simulink model "AFC_FFNN_trainbfg_15_15_15_15_Nor_July_15"  (R2021a)
settings: Solver=ode15s  StartTime=0.0  StopTime=T  MaxStep=.01  RelTol=1e-3
undefined symbols (not defined in the file): AF_sensor_tol, fault_time, fuel_inj_tol, kappa_tol, MAF_sensor_tol, pump_tol, tau_ww_tol, x_gain, x_offset, y_gain, y_offset
libraries: neural x66
(part 3 of 3)

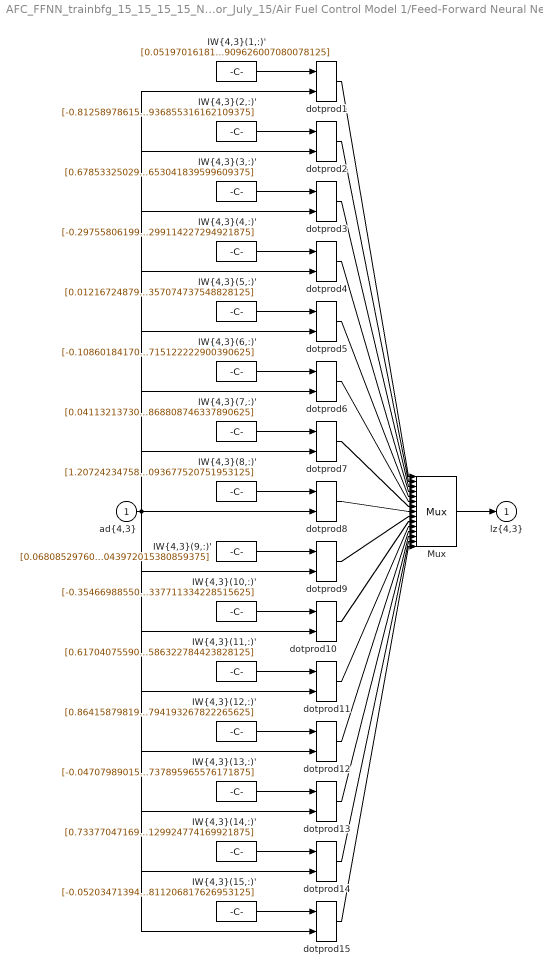
== system AFC_FFNN_trainbfg_15_15_15_15_Nor_July_15/Air Fuel Control Model 1/Feed-Forward Neural Network/Layer 4/LW{4,3} ==
  "ad{4,3}" : Inport  PortDimensions=15
      mask Display: e = 0.06;c1 = [120 230 180]/255;c2 = ([120 230 180]+0)/(256+128);c3 = ([120 230 180]+128)/(256+128);patch([0 1 1 0],[0 0 1 1],c1);patch([0 1 1 1-e 1-e 0+e],[0 0 1 1-e 0+e 0+e],c2);patch([0 0 1 1-e 0+e 0+e],[0 1 1 1-e 1-e 0+e],c3);plot([0 1 1 0 0],[0 0 1 1 0]);
  "IW{4,3}(1,:)'" : Constant  Value=[0.051970161810708959126969830322195775806903839111328125;-0.126328957419962417674241805798374116420745849609375;0.9965377844405078899825412008794955909252166748046875;0.1675357955800376164035014880937524139881134033203125;0.404152985833085953704113535422948189079761505126953125;0.86478973592762808930700657583656720817089080810546875;0.518227264629068873347250701044686138629913330078125;0.2715980210299460129164117461186833679676055908203125;-0.651185893458846809522810872294940054416656494140625;0.319204255476944143143924748073914088308811187744140625;-0.2569115041239822261331937625072896480560302734375;0.057105623983778171226521891412630793638527393341064453125;0.1070777617804902492881780062816687859594821929931640625;-0.82642827178341027316577083183801732957363128662109375;-0.0287179233202064232433059487448190338909626007080078125]
      mask Display: e = 0.06;c1 = [120 150 230]/255;c2 = ([120 150 230]+0)/383;c3 = ([120 150 230]+128)/383;patch([0 1 1 0],[0 0 1 1],c1);patch([0 1 1 1-e 1-e 0+e],[0 0 1 1-e 0+e 0+e],c2);patch([0 0 1 1-e 0+e 0+e],[0 1 1 1-e 1-e 0+e],c3);plot([0 1 1 0 0],[0 0 1 1 0]);disp('weights');
  "IW{4,3}(10,:)'" : Constant  Value=[-0.354669885508523241579581508631235919892787933349609375;-0.77194952346326062286863134431769140064716339111328125;-0.81601175837494732689947340986691415309906005859375;0.379241236877119636261568302870728075504302978515625;-0.3569337623701613892990280874073505401611328125;-0.792692853946006525944767417968250811100006103515625;-0.14953643024327778476845196564681828022003173828125;-0.0850888851491766740053890316630713641643524169921875;-0.9650803191481467369072788642370142042636871337890625;0.405282382043266498072853210032917559146881103515625;0.49853527113881723753507912988425232470035552978515625;0.271502161657881657674806774593889713287353515625;0.3751637008352275426403821256826631724834442138671875;0.8806065157679683341740428659250028431415557861328125;-0.59715081395340219305722939679981209337711334228515625]
      mask Display: e = 0.06;c1 = [120 150 230]/255;c2 = ([120 150 230]+0)/383;c3 = ([120 150 230]+128)/383;patch([0 1 1 0],[0 0 1 1],c1);patch([0 1 1 1-e 1-e 0+e],[0 0 1 1-e 0+e 0+e],c2);patch([0 0 1 1-e 0+e 0+e],[0 1 1 1-e 1-e 0+e],c3);plot([0 1 1 0 0],[0 0 1 1 0]);disp('weights');
  "IW{4,3}(11,:)'" : Constant  Value=[0.617040755904621818217492545954883098602294921875;0.700604235086529580911474113236181437969207763671875;0.511371924663512888997729533002711832523345947265625;0.08963480551315772260068115429021418094635009765625;-0.165964035301581269710169408426736481487751007080078125;0.5031390236482307098953015156439505517482757568359375;0.6633082060229267273854247832787223160266876220703125;-0.709798207981374940089835945400409400463104248046875;0.831096977986841789487471032771281898021697998046875;-0.4122922604000514024136236912454478442668914794921875;-0.0723067339924330365619198346394114196300506591796875;-0.376003397439505893107281053744372911751270294189453125;0.1695995889177781823509150171958026476204395294189453125;0.90183804417739477088389321579597890377044677734375;-1.10240234673867565362570530851371586322784423828125]
      mask Display: e = 0.06;c1 = [120 150 230]/255;c2 = ([120 150 230]+0)/383;c3 = ([120 150 230]+128)/383;patch([0 1 1 0],[0 0 1 1],c1);patch([0 1 1 1-e 1-e 0+e],[0 0 1 1-e 0+e 0+e],c2);patch([0 0 1 1-e 0+e 0+e],[0 1 1 1-e 1-e 0+e],c3);plot([0 1 1 0 0],[0 0 1 1 0]);disp('weights');
  "IW{4,3}(12,:)'" : Constant  Value=[0.86415879819654961568886619716067798435688018798828125;0.1203834479508809618408804453792981803417205810546875;0.133982984467660326544091731193475425243377685546875;-0.0193712548926814331906598454224877059459686279296875;-0.1402303904538838852378290766864665783941745758056640625;1.0897626729878930884609644635929726064205169677734375;0.67839995473971459460926780593581497669219970703125;-0.7508734295524204238603260819218121469020843505859375;0.0334637355957545512552542277262546122074127197265625;0.87659168440380941245138046724605374038219451904296875;-0.980282012415287784534712045569904148578643798828125;0.8080715194356573594092196799465455114841461181640625;-0.76798820148797342088897721623652614653110504150390625;-0.313277713257333612073551876164856366813182830810546875;0.35824559123448074249296269044862128794193267822265625]
      mask Display: e = 0.06;c1 = [120 150 230]/255;c2 = ([120 150 230]+0)/383;c3 = ([120 150 230]+128)/383;patch([0 1 1 0],[0 0 1 1],c1);patch([0 1 1 1-e 1-e 0+e],[0 0 1 1-e 0+e 0+e],c2);patch([0 0 1 1-e 0+e 0+e],[0 1 1 1-e 1-e 0+e],c3);plot([0 1 1 0 0],[0 0 1 1 0]);disp('weights');
  "IW{4,3}(13,:)'" : Constant  Value=[-0.04707989015845824576356193347237422131001949310302734375;-0.74905307149987765402698869365849532186985015869140625;0.5757676864781038350571407136158086359500885009765625;0.71306953158993646724184145568870007991790771484375;-0.5913842257991495099389567258185707032680511474609375;-0.37587419944126232440595458683674223721027374267578125;-0.336733940480412829998613233328796923160552978515625;-0.004068794637174466544138340395875275135040283203125;0.0693886439127837650886476694722659885883331298828125;0.05129647141780004082622923533563152886927127838134765625;-0.0307644877411348029172533102837405749596655368804931640625;-0.334572257247817306247128499308018945157527923583984375;0.2420501582242300664393752640535240061581134796142578125;-0.77793738892486985481156125388224609196186065673828125;1.190993380582610949858235471765510737895965576171875]
      mask Display: e = 0.06;c1 = [120 150 230]/255;c2 = ([120 150 230]+0)/383;c3 = ([120 150 230]+128)/383;patch([0 1 1 0],[0 0 1 1],c1);patch([0 1 1 1-e 1-e 0+e],[0 0 1 1-e 0+e 0+e],c2);patch([0 0 1 1-e 0+e 0+e],[0 1 1 1-e 1-e 0+e],c3);plot([0 1 1 0 0],[0 0 1 1 0]);disp('weights');
  "IW{4,3}(14,:)'" : Constant  Value=[0.73377047169310072316505966227850876748561859130859375;0.59318557483826050980013633306953124701976776123046875;0.97198033802115357815409879549406468868255615234375;-0.6828295214165047699594879304640926420688629150390625;-0.727325596267671681260935656609944999217987060546875;-0.007302479939687057074182430227438089787028729915618896484375;-0.74322529652487201445865139248780906200408935546875;0.2139264100071509577816186720156110823154449462890625;0.7427593592867605121199403583887033164501190185546875;-0.6586018858724387303738012633402831852436065673828125;-0.1654446667255996816781049574274220503866672515869140625;0.46870267206282634209202342390199191868305206298828125;-0.2075915391437903878557591497155954129993915557861328125;0.271907738610796367861865974191459827125072479248046875;-0.1551503657733785679351257158486987464129924774169921875]
      mask Display: e = 0.06;c1 = [120 150 230]/255;c2 = ([120 150 230]+0)/383;c3 = ([120 150 230]+128)/383;patch([0 1 1 0],[0 0 1 1],c1);patch([0 1 1 1-e 1-e 0+e],[0 0 1 1-e 0+e 0+e],c2);patch([0 0 1 1-e 0+e 0+e],[0 1 1 1-e 1-e 0+e],c3);plot([0 1 1 0 0],[0 0 1 1 0]);disp('weights');
  "IW{4,3}(15,:)'" : Constant  Value=[-0.052034713940864042724943061557496548630297183990478515625;0.7331140203109469677400511500309221446514129638671875;0.134145500728414412972000491208746097981929779052734375;0.14154267621595284509794510086067020893096923828125;0.2930468609746219588174653836176730692386627197265625;0.4199159074445060202407375982147641479969024658203125;-0.93186243047858141608230653218924999237060546875;0.04270707824443764621946684201247990131378173828125;0.350319910837068260178739365073852241039276123046875;-0.342224755301396121875967537562246434390544891357421875;0.12252060779661462508460800790999201126396656036376953125;0.253549817145111544558488958500674925744533538818359375;0.89990162781650495649188314928323961794376373291015625;0.9157133079961587984740845058695413172245025634765625;-0.55171023855309730965501557875541038811206817626953125]
      mask Display: e = 0.06;c1 = [120 150 230]/255;c2 = ([120 150 230]+0)/383;c3 = ([120 150 230]+128)/383;patch([0 1 1 0],[0 0 1 1],c1);patch([0 1 1 1-e 1-e 0+e],[0 0 1 1-e 0+e 0+e],c2);patch([0 0 1 1-e 0+e 0+e],[0 1 1 1-e 1-e 0+e],c3);plot([0 1 1 0 0],[0 0 1 1 0]);disp('weights');
  "IW{4,3}(2,:)'" : Constant  Value=[-0.8125897861595652305055637043551541864871978759765625;0.6696301702838931557693058493896387517452239990234375;0.0494682777685733210404350757016800343990325927734375;0.817877680294583964126786668202839791774749755859375;0.148708664585286864934232653467915952205657958984375;-0.1140448432503557985029374322039075195789337158203125;0.2540073049131656990340388801996596157550811767578125;-0.0952829278543816382551767674158327281475067138671875;-0.869787452715599318509021031786687672138214111328125;0.0628607068926652079454697741311974823474884033203125;-0.99548355810059963033609164995141327381134033203125;0.7449122353879769065088112256489694118499755859375;0.54699886858855517601796236704103648662567138671875;-0.6575546792262390027872243081219494342803955078125;-0.1118978718546799200339592061936855316162109375]
      mask Display: e = 0.06;c1 = [120 150 230]/255;c2 = ([120 150 230]+0)/383;c3 = ([120 150 230]+128)/383;patch([0 1 1 0],[0 0 1 1],c1);patch([0 1 1 1-e 1-e 0+e],[0 0 1 1-e 0+e 0+e],c2);patch([0 0 1 1-e 0+e 0+e],[0 1 1 1-e 1-e 0+e],c3);plot([0 1 1 0 0],[0 0 1 1 0]);disp('weights');
  "IW{4,3}(3,:)'" : Constant  Value=[0.67853325029204014651185161710600368678569793701171875;0.649225618879884169842853225418366491794586181640625;0.0244182303058833767572810558021956239826977252960205078125;0.91905635318846368164713567239232361316680908203125;0.0660607060368446907805406453917385078966617584228515625;-0.11251524592039625904948962897833553142845630645751953125;0.0515896481136202122996792240883223712444305419921875;-0.5706344744726050688399254795513115823268890380859375;0.543627018010135909520386121585033833980560302734375;-0.718405788341949236297523384564556181430816650390625;0.072829230863325822298293132917024195194244384765625;1.1098893041941300108277346225804649293422698974609375;-0.6268628150142021571156192294438369572162628173828125;0.64965362929718917239796383000793866813182830810546875;0.24955078029045585363832060465938411653041839599609375]
      mask Display: e = 0.06;c1 = [120 150 230]/255;c2 = ([120 150 230]+0)/383;c3 = ([120 150 230]+128)/383;patch([0 1 1 0],[0 0 1 1],c1);patch([0 1 1 1-e 1-e 0+e],[0 0 1 1-e 0+e 0+e],c2);patch([0 0 1 1-e 0+e 0+e],[0 1 1 1-e 1-e 0+e],c3);plot([0 1 1 0 0],[0 0 1 1 0]);disp('weights');
  "IW{4,3}(4,:)'" : Constant  Value=[-0.2975580619978703822425813996233046054840087890625;0.216290439667084388730700084124691784381866455078125;-0.532417130550156603163713953108526766300201416015625;-0.9093614745271327848286091466434299945831298828125;-0.4789695686043524691655193237238563597202301025390625;-0.2897506116045913682199852701160125434398651123046875;-0.09180504603758521398049197159707546234130859375;0.0106020674426960948011355867492966353893280029296875;-0.661658236974961067033973449724726378917694091796875;0.659602628583194405820222527836449444293975830078125;-0.1565907405649149541915221561794169247150421142578125;0.1760495719019183891163038424565456807613372802734375;-0.4251169390202733655570455084671266376972198486328125;-0.2251245296180972577104739684727974236011505126953125;-0.4908767677254395334074388301814906299114227294921875]
      mask Display: e = 0.06;c1 = [120 150 230]/255;c2 = ([120 150 230]+0)/383;c3 = ([120 150 230]+128)/383;patch([0 1 1 0],[0 0 1 1],c1);patch([0 1 1 1-e 1-e 0+e],[0 0 1 1-e 0+e 0+e],c2);patch([0 0 1 1-e 0+e 0+e],[0 1 1 1-e 1-e 0+e],c3);plot([0 1 1 0 0],[0 0 1 1 0]);disp('weights');
  "IW{4,3}(5,:)'" : Constant  Value=[0.0121672487908398678502219780739324050955474376678466796875;-0.279291635237711555195261325934552587568759918212890625;0.39580478815836916961501401601708494126796722412109375;-0.41888196527845256156297182315029203891754150390625;0.96026476375696512288726580663933418691158294677734375;-0.07705788414508407679903712050872854888439178466796875;-0.7369962098884264012355060913250781595706939697265625;-0.641380277290782174759442568756639957427978515625;-0.1470570579484429263317224467755295336246490478515625;-0.552357426018287522850869208923541009426116943359375;0.5426753535136719097664581568096764385700225830078125;-0.6534036514741854428933720555505715310573577880859375;0.8952196061710460117666343649034388363361358642578125;-0.71648872638311933425114830242819152772426605224609375;1.101038667785545488442267014761455357074737548828125]
      mask Display: e = 0.06;c1 = [120 150 230]/255;c2 = ([120 150 230]+0)/383;c3 = ([120 150 230]+128)/383;patch([0 1 1 0],[0 0 1 1],c1);patch([0 1 1 1-e 1-e 0+e],[0 0 1 1-e 0+e 0+e],c2);patch([0 0 1 1-e 0+e 0+e],[0 1 1 1-e 1-e 0+e],c3);plot([0 1 1 0 0],[0 0 1 1 0]);disp('weights');
  "IW{4,3}(6,:)'" : Constant  Value=[-0.10860184170805009529203744023106992244720458984375;0.0194190021120725919701044404064305126667022705078125;0.7664594013744976397362052011885680258274078369140625;-0.0669174495247097933514623946393840014934539794921875;-0.69434533003424991903784757596440613269805908203125;-0.8237276518362877109069586367695592343807220458984375;0.2052424366817493517345383224892430007457733154296875;-0.252655580676456548161468163016252219676971435546875;0.66723256757870075261962483637034893035888671875;0.957094387199472595995075607788749039173126220703125;-0.3538932796519895784825848750188015401363372802734375;-0.7059302300365530857817475407500751316547393798828125;-0.8348335978485235120416518839192576706409454345703125;-0.00859368877235322514707149821333587169647216796875;-0.1199812481452335877207815428846515715122222900390625]
      mask Display: e = 0.06;c1 = [120 150 230]/255;c2 = ([120 150 230]+0)/383;c3 = ([120 150 230]+128)/383;patch([0 1 1 0],[0 0 1 1],c1);patch([0 1 1 1-e 1-e 0+e],[0 0 1 1-e 0+e 0+e],c2);patch([0 0 1 1-e 0+e 0+e],[0 1 1 1-e 1-e 0+e],c3);plot([0 1 1 0 0],[0 0 1 1 0]);disp('weights');
  "IW{4,3}(7,:)'" : Constant  Value=[0.041132137300131328683239217980371904559433460235595703125;-0.8170410050061052142922335406183265149593353271484375;0.880640458053120855907991426647640764713287353515625;-0.8672502897025411439102526856004260480403900146484375;0.375021567196341221173128133159480057656764984130859375;0.74060605087412023639359404114657081663608551025390625;0.208223727655667989466792278108187019824981689453125;0.4991232146158661731050187881919555366039276123046875;0.8040042399321531974010213161818683147430419921875;-0.9287241362211251516356469437596388161182403564453125;-0.2369142647526545075731263523266534321010112762451171875;-0.381204863194875620546753225426073186099529266357421875;-0.8032444535196681112410033165360800921916961669921875;0.3691943099448593557099229656159877777099609375;0.0186137077896842174917768630848513566888868808746337890625]
      mask Display: e = 0.06;c1 = [120 150 230]/255;c2 = ([120 150 230]+0)/383;c3 = ([120 150 230]+128)/383;patch([0 1 1 0],[0 0 1 1],c1);patch([0 1 1 1-e 1-e 0+e],[0 0 1 1-e 0+e 0+e],c2);patch([0 0 1 1-e 0+e 0+e],[0 1 1 1-e 1-e 0+e],c3);plot([0 1 1 0 0],[0 0 1 1 0]);disp('weights');
  "IW{4,3}(8,:)'" : Constant  Value=[1.2072423475886087107511457361397333443164825439453125;-0.11524115643226974514679028516184189356863498687744140625;0.34222553991496285075157857136218808591365814208984375;0.3645259514743426354499433728051371872425079345703125;0.339188479923518582115349317973596043884754180908203125;-0.42353456120008792229469918311224319040775299072265625;0.724771462281134315475128460093401372432708740234375;-0.6004800474653737563102140484261326491832733154296875;-0.4151526394563258559600171793135814368724822998046875;-0.338141381416675101956315074858139269053936004638671875;0.66970817401589821660223833532654680311679840087890625;-1.143557580187915423408639981062151491641998291015625;-0.2154730791377687804111218383695813827216625213623046875;0.418907292844881318227834299250389449298381805419921875;-0.23972582973012468432472132917609997093677520751953125]
      mask Display: e = 0.06;c1 = [120 150 230]/255;c2 = ([120 150 230]+0)/383;c3 = ([120 150 230]+128)/383;patch([0 1 1 0],[0 0 1 1],c1);patch([0 1 1 1-e 1-e 0+e],[0 0 1 1-e 0+e 0+e],c2);patch([0 0 1 1-e 0+e 0+e],[0 1 1 1-e 1-e 0+e],c3);plot([0 1 1 0 0],[0 0 1 1 0]);disp('weights');
  "IW{4,3}(9,:)'" : Constant  Value=[0.068085297603662386922707128178444691002368927001953125;-0.2575471222895735490254764954443089663982391357421875;-0.59973830245885439982345133103081025183200836181640625;0.77825576456782386003396823070943355560302734375;0.2305592100961315893403735799438436515629291534423828125;-0.57777072238661719705277164393919520080089569091796875;-0.748255587499393026718053079093806445598602294921875;-0.8930452997856173080748476422741077840328216552734375;-0.3068847913407621863512986237765289843082427978515625;0.5477080755002823320154448083485476672649383544921875;-0.98925761512351118032171370941796340048313140869140625;-0.64119907846262014228244652258581481873989105224609375;-0.41004655161942349383963346554082818329334259033203125;-0.2154503146029320415077989991914364509284496307373046875;-1.275394006992440321113235768279992043972015380859375]
      mask Display: e = 0.06;c1 = [120 150 230]/255;c2 = ([120 150 230]+0)/383;c3 = ([120 150 230]+128)/383;patch([0 1 1 0],[0 0 1 1],c1);patch([0 1 1 1-e 1-e 0+e],[0 0 1 1-e 0+e 0+e],c2);patch([0 0 1 1-e 0+e 0+e],[0 1 1 1-e 1-e 0+e],c3);plot([0 1 1 0 0],[0 0 1 1 0]);disp('weights');
  Mux : Mux  Inputs=15
      mask Display: e = 0.06;c1 = [120 150 230]/255;c2 = ([120 150 230]+0)/383;c3 = ([120 150 230]+128)/383;patch([0 1 1 0],[0 0 1 1],c1);patch([0 1 1 1-e 1-e 0+e],[0 0 1 1-e 0+e 0+e],c2);patch([0 0 1 1-e 0+e 0+e],[0 1 1 1-e 1-e 0+e],c3);plot([0 1 1 0 0],[0 0 1 1 0]);disp('Mux');
  dotprod{1..15} (15 alike) : neural/Weight Functions/dotprod
  "lz{4,3}" : Outport
      mask Display: e = 0.06;c1 = [120 230 180]/255;c2 = ([120 230 180]+0)/(256+128);c3 = ([120 230 180]+128)/(256+128);patch([0 1 1 0],[0 0 1 1],c1);patch([0 1 1 1-e 1-e 0+e],[0 0 1 1-e 0+e 0+e],c2);patch([0 0 1 1-e 0+e 0+e],[0 1 1 1-e 1-e 0+e],c3);plot([0 1 1 0 0],[0 0 1 1 0]);
  wires:
  Mux/1 -> "lz{4,3}"/1
  dotprod15/1 -> Mux/15
  "IW{4,3}(15,:)'"/1 -> dotprod15/1
  dotprod14/1 -> Mux/14
  "IW{4,3}(14,:)'"/1 -> dotprod14/1
  dotprod13/1 -> Mux/13
  "IW{4,3}(13,:)'"/1 -> dotprod13/1
  dotprod12/1 -> Mux/12
  "IW{4,3}(12,:)'"/1 -> dotprod12/1
  dotprod11/1 -> Mux/11
  "IW{4,3}(11,:)'"/1 -> dotprod11/1
  dotprod10/1 -> Mux/10
  "IW{4,3}(10,:)'"/1 -> dotprod10/1
  dotprod9/1 -> Mux/9
  "IW{4,3}(9,:)'"/1 -> dotprod9/1
  dotprod8/1 -> Mux/8
  "IW{4,3}(8,:)'"/1 -> dotprod8/1
  dotprod7/1 -> Mux/7
  "IW{4,3}(7,:)'"/1 -> dotprod7/1
  dotprod6/1 -> Mux/6
  "IW{4,3}(6,:)'"/1 -> dotprod6/1
  dotprod5/1 -> Mux/5
  "IW{4,3}(5,:)'"/1 -> dotprod5/1
  dotprod4/1 -> Mux/4
  "IW{4,3}(4,:)'"/1 -> dotprod4/1
  dotprod3/1 -> Mux/3
  "IW{4,3}(3,:)'"/1 -> dotprod3/1
  dotprod2/1 -> Mux/2
  "IW{4,3}(2,:)'"/1 -> dotprod2/1
  dotprod1/1 -> Mux/1
  "ad{4,3}"/1 -> dotprod15/2, dotprod14/2, dotprod13/2, dotprod12/2, dotprod11/2, dotprod10/2, dotprod9/2, dotprod8/2, dotprod7/2, dotprod6/2, dotprod5/2, dotprod4/2, dotprod3/2, dotprod2/2, dotprod1/2
  "IW{4,3}(1,:)'"/1 -> dotprod1/1

== system AFC_FFNN_trainbfg_15_15_15_15_Nor_July_15/Air Fuel Control Model 1/Feed-Forward Neural Network/Layer 5/Delays 1 ==
  "p{5}" : Inport  PortDimensions=15
      mask Display: e = 0.06;c1 = [120 230 180]/255;c2 = ([120 230 180]+0)/(256+128);c3 = ([120 230 180]+128)/(256+128);patch([0 1 1 0],[0 0 1 1],c1);patch([0 1 1 1-e 1-e 0+e],[0 0 1 1-e 0+e 0+e],c2);patch([0 0 1 1-e 0+e 0+e],[0 1 1 1-e 1-e 0+e],c3);plot([0 1 1 0 0],[0 0 1 1 0]);
  mux : Mux  Inputs=1
      mask Display: e = 0.06;c1 = [120 150 230]/255;c2 = ([120 150 230]+0)/383;c3 = ([120 150 230]+128)/383;patch([0 1 1 0],[0 0 1 1],c1);patch([0 1 1 1-e 1-e 0+e],[0 0 1 1-e 0+e 0+e],c2);patch([0 0 1 1-e 0+e 0+e],[0 1 1 1-e 1-e 0+e],c3);plot([0 1 1 0 0],[0 0 1 1 0]);disp('Mux')
  "pd{5,4}" : Outport
      mask Display: e = 0.06;c1 = [120 230 180]/255;c2 = ([120 230 180]+0)/(256+128);c3 = ([120 230 180]+128)/(256+128);patch([0 1 1 0],[0 0 1 1],c1);patch([0 1 1 1-e 1-e 0+e],[0 0 1 1-e 0+e 0+e],c2);patch([0 0 1 1-e 0+e 0+e],[0 1 1 1-e 1-e 0+e],c3);plot([0 1 1 0 0],[0 0 1 1 0]);
  wires:
  mux/1 -> "pd{5,4}"/1
  "p{5}"/1 -> mux/1

== system AFC_FFNN_trainbfg_15_15_15_15_Nor_July_15/Air Fuel Control Model 1/Feed-Forward Neural Network/Layer 5/LW{5,4} ==
  "ad{5,4}" : Inport  PortDimensions=15
      mask Display: e = 0.06;c1 = [120 230 180]/255;c2 = ([120 230 180]+0)/(256+128);c3 = ([120 230 180]+128)/(256+128);patch([0 1 1 0],[0 0 1 1],c1);patch([0 1 1 1-e 1-e 0+e],[0 0 1 1-e 0+e 0+e],c2);patch([0 0 1 1-e 0+e 0+e],[0 1 1 1-e 1-e 0+e],c3);plot([0 1 1 0 0],[0 0 1 1 0]);
  "IW{5,4}(1,:)'" : Constant  Value=[0.63232546415590906718762198579497635364532470703125;-0.169051723874596770968992132111452519893646240234375;-0.69946240155650063474723765466478653252124786376953125;0.459821670027029227867387817241251468658447265625;0.39674119614733693861552410453441552817821502685546875;-0.9852702587518942234368068966432474553585052490234375;-0.338339474410549456706576165743172168731689453125;0.474516192083134058510296426902641542255878448486328125;0.33806496686015063968255844883969984948635101318359375;0.1484491629542154245147145275041111744940280914306640625;0.229695058132312557308551959067699499428272247314453125;1.7530956139152760187016610871069133281707763671875;0.716214319281081035484248786815442144870758056640625;-0.150907167366728989232882440774119459092617034912109375;0.273084464625173328755636248388327658176422119140625]
      mask Display: e = 0.06;c1 = [120 150 230]/255;c2 = ([120 150 230]+0)/383;c3 = ([120 150 230]+128)/383;patch([0 1 1 0],[0 0 1 1],c1);patch([0 1 1 1-e 1-e 0+e],[0 0 1 1-e 0+e 0+e],c2);patch([0 0 1 1-e 0+e 0+e],[0 1 1 1-e 1-e 0+e],c3);plot([0 1 1 0 0],[0 0 1 1 0]);disp('weights');
  Mux : Mux  Inputs=1
      mask Display: e = 0.06;c1 = [120 150 230]/255;c2 = ([120 150 230]+0)/383;c3 = ([120 150 230]+128)/383;patch([0 1 1 0],[0 0 1 1],c1);patch([0 1 1 1-e 1-e 0+e],[0 0 1 1-e 0+e 0+e],c2);patch([0 0 1 1-e 0+e 0+e],[0 1 1 1-e 1-e 0+e],c3);plot([0 1 1 0 0],[0 0 1 1 0]);disp('Mux');
  dotprod1 : neural/Weight Functions/dotprod
  "lz{5,4}" : Outport
      mask Display: e = 0.06;c1 = [120 230 180]/255;c2 = ([120 230 180]+0)/(256+128);c3 = ([120 230 180]+128)/(256+128);patch([0 1 1 0],[0 0 1 1],c1);patch([0 1 1 1-e 1-e 0+e],[0 0 1 1-e 0+e 0+e],c2);patch([0 0 1 1-e 0+e 0+e],[0 1 1 1-e 1-e 0+e],c3);plot([0 1 1 0 0],[0 0 1 1 0]);
  wires:
  Mux/1 -> "lz{5,4}"/1
  dotprod1/1 -> Mux/1
  "ad{5,4}"/1 -> dotprod1/2
  "IW{5,4}(1,:)'"/1 -> dotprod1/1
